simulink model "FOCsimulation"  (R2023b)
settings: Solver=VariableStepAuto  StartTime=0.0  StopTime=12  RelTol=1e-3
values from neighbouring files (symbols this model uses):
  acceleration = 20000/PU_System.N_base    [FOC_Script.m]    (also in Motor_script.m)
  PI_params = mcb.internal.SetControllerParameters(pmsm,inverter,PU_System,T_pwm,2*Ts,Ts_speed)    [FOC_Script.m]    (also in Motor_script.m)
  Speed_openLoop_PU = 0.1    [FOC_Script.m]    (also in Motor_script.m)
  T_Ref_openLoop = 1    [FOC_Script.m]    (also in Motor_script.m)
  Ts = T_pwm    (= 0.0001)    [FOC_Script.m]    (also in Motor_script.m = 3.33333333333e-05)
  Ts_motor = T_pwm/2    (= 5e-05)    [FOC_Script.m]    (also in Motor_script.m = 1.66666666667e-05)
  Ts_speed = 30*Ts    (= 0.003)    [FOC_Script.m]    (also in Motor_script.m = 0.001)
undefined symbols (not defined in the file or in its folder): inverter, pmsm, PU_System, sigbuilder_block, target
libraries: mcbcontrolslib x11, slpidlib x3, mcbpositiondecoderlib x2, simulink x1, dspsrcs4 x1, mcbplantlib x1, autolibpmsmexterior x1
(part 2 of 2)

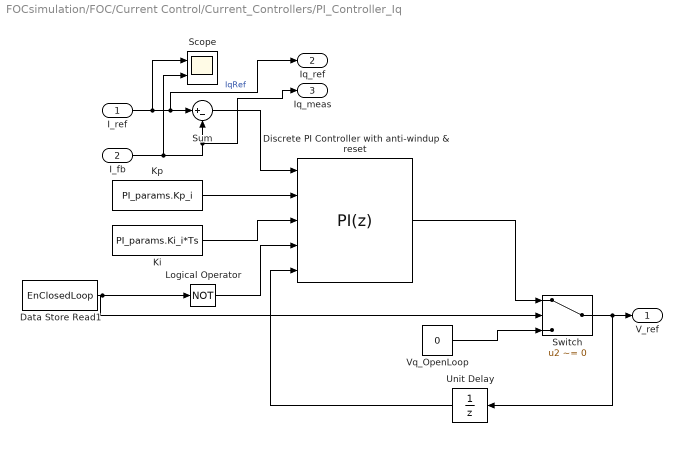
== system FOCsimulation/FOC/Current Control/Current_Controllers/PI_Controller_Iq ==
  I_ref : Inport
  I_fb : Inport  Port=2
  Data Store Read1 : DataStoreRead  DataStoreName=EnClosedLoop  IndexOptions=Index vector (dialog)  Indices=1  OutputSizes=1
  Discrete PI Controller with anti-windup & reset : slpidlib/PID Controller  Controller=PI  Form=Parallel  TimeDomain=Discrete-time  UseExternalTs=off  SampleTime=-1  IntegratorMethod=Forward Euler  FilterMethod=Forward Euler  ControllerParametersSource=external  P=1  I=1  UseKiTs=on  D=0  N=100  UseFilter=on  TunerSelectOption=Transfer Function Based (PID Tuner App)  InitialConditionSource=external  InitialConditionForIntegrator=0  InitialConditionForFilter=0  DifferentiatorICPrevScaledInput=0  ExternalReset=level  TrackingMode=off  Kt=1  LimitOutput=on  SatLimitsSource=internal  UpperSaturationLimit=1  LowerSaturationLimit=-1  LinearizeAsGain=on  AntiWindupMode=clamping  Kb=1  LimitIntegrator=off  UpperIntegratorSaturationLimit=inf  LowerIntegratorSaturationLimit=-inf  RndMeth=Simplest  POutMin=[]  POutMax=[]  IOutMin=[]  IOutMax=[]  DOutMin=[]  DOutMax=[]  NOutMin=[]  NOutMax=[]  SumOutMin=[]  SumOutMax=[]  SaturationOutDataTypeStr=Inherit: Inherit via back propagation  SaturationOutMin=[]  SaturationOutMax=[]  PParamMin=[]  PParamMax=[]  IParamMin=[]  IParamMax=[]  DParamMin=[]  DParamMax=[]  NParamMin=[]  NParamMax=[]  KbParamMin=[]  KbParamMax=[]  KtParamMin=[]  KtParamMax=[]  KbOutMin=[]  KbOutMax=[]  KtOutMin=[]  KtOutMax=[]  IntegratorOutMin=[]  IntegratorOutMax=[]  FilterOutMin=[]  FilterOutMax=[]  SumI1OutMin=[]  SumI1OutMax=[]  SumI2OutMin=[]  SumI2OutMax=[]  SumI3OutMin=[]  SumI3OutMax=[]  SumI4OutMin=[]  SumI4OutMax=[]  SumDOutMin=[]  SumDOutMax=[]  DifferentiatorOutMin=[]  DifferentiatorOutMax=[]  FilterDiffOutCoefMin=[]  FilterDiffOutCoefMax=[]  ReciprocalOutMin=[]  ReciprocalOutMax=[]  SumDenOutMin=[]  SumDenOutMax=[]  SumNumOutMin=[]  SumNumOutMax=[]  DivideOutMin=[]  DivideOutMax=[]  UdiffTsProdOutMin=[]  UdiffTsProdOutMax=[]  NTsProdOutMin=[]  NTsProdOutMax=[]  UintegralTsProdOutMin=[]  UintegralTsProdOutMax=[]  UngainTsProdOutMin=[]  UngainTsProdOutMax=[]  ClampingZeroOutDataTypeStr=Inherit: Inherit via back propagation  ClampingZeroOutMin=[]  ClampingZeroOutMax=[]  FilterDenConstantOutDataTypeStr=Inherit: Inherit via back propagation  FilterDenConstantOutMin=[]  FilterDenConstantOutMax=[]  PCopyOutDataTypeStr=Inherit: Inherit via back propagation  PCopyOutMin=[]  PCopyOutMax=[]  NCopyOutDataTypeStr=Inherit: Inherit via back propagation  NCopyOutMin=[]  NCopyOutMax=[]  IntegratorContinuousStateAttributes=''  IntegratorStateMustResolveToSignalObject=off  IntegratorRTWStateStorageClass=Auto  FilterContinuousStateAttributes=''  FilterStateMustResolveToSignalObject=off  FilterRTWStateStorageClass=Auto  ParallelPVariant=ExternalParameters  IdealPVariant=Disabled  IVariant=ExternalParameters  DVariant=Disabled  IntegratorVariant=Discrete  SatVariant=Enabled  AWVariant=DiscClampingParallel  PCopyVariant=Disabled  TRVariant=Disabled  FdbkBlocksVariant=Forward  IdealPFdbkVariant=Disabled  SatFdbkVariant=Disabled  DerivativeFilterVariant=Disabled  NVariant=Disabled  NCopyVariant=Disabled_SignalSpec  FilterICVariant=Disabled  IntegratorICVariant=ExternalICs  ExternalResetVariant=ExternalReset  TRSumVariant=Passthrough  SumFdbkVariant=Disabled  SumVariant=Sum_PI  TsampFilterVariant=InternalTs  TsampNgainVariant=Passthrough  TsampIntegralVariant=Disabled_SignalSpec  ExternalSaturationOutDataTypeStr=Inherit: Same as second input
      settings: LibrarySourceBlock=mcbcontrolslib/PI Controller
  Ki : Constant  Value=PI_params.Ki_i*Ts  OutDataTypeStr=dataType  SampleTime=-1
  Kp : Constant  Value=PI_params.Kp_i  OutDataTypeStr=dataType  SampleTime=-1
  Logical Operator : Logic  Operator=NOT  IconShape=distinctive  AllPortsSameDT=off  OutDataTypeStr=boolean
  Scope : Scope  NumInputPorts=2
  Sum : Sum  Inputs=|+-  OutDataTypeStr=Inherit: Same as first input
  Switch : Switch  Criteria=u2 ~= 0  RndMeth=Simplest  SaturateOnIntegerOverflow=off  InputSameDT=off
  Unit Delay : UnitDelay  SampleTime=-1  HasFrameUpgradeWarning=on
  Vq_OpenLoop : Constant  Value=0  OutDataTypeStr=dataType  SampleTime=-1
  V_ref : Outport  VectorParamsAs1DForOutWhenUnconnected=off
  Iq_ref : Outport  Port=2  VectorParamsAs1DForOutWhenUnconnected=off
  Iq_meas : Outport  Port=3  VectorParamsAs1DForOutWhenUnconnected=off
  wires:
  Switch/1 -> V_ref/1, Unit Delay/1
  I_fb/1 -> Scope/2, Iq_meas/1, Sum/2
  Sum/1 -> Discrete PI Controller with anti-windup & reset/1
  Kp/1 -> Discrete PI Controller with anti-windup & reset/2
  I_ref/1 -> Scope/1, Iq_ref/1, Sum/1  "IqRef"
  Ki/1 -> Discrete PI Controller with anti-windup & reset/3
  Logical Operator/1 -> Discrete PI Controller with anti-windup & reset/4
  Unit Delay/1 -> Discrete PI Controller with anti-windup & reset/5
  Discrete PI Controller with anti-windup & reset/1 -> Switch/1
  Vq_OpenLoop/1 -> Switch/3
  Data Store Read1/1 -> Switch/2, Logical Operator/1

== system FOCsimulation/FOC/Speed Control/Speed_Ref_Selector/Absolute value ==
  Speed_Ref : Inport
  Rate Limiter : RateLimiter  RisingSlewLimit=acceleration  FallingSlewLimit=-acceleration  SampleTimeMode=inherited  InitialCondition=Speed_openLoop_PU
  Rate Limiter1 : RateLimiter  RisingSlewLimit=acceleration  FallingSlewLimit=-acceleration  SampleTimeMode=inherited  InitialCondition=-Speed_openLoop_PU
  Switch : Switch  SaturateOnIntegerOverflow=off  InputSameDT=off
  Out1 : Outport
  wires:
  Switch/1 -> Out1/1
  Rate Limiter/1 -> Switch/1
  Rate Limiter1/1 -> Switch/3
  Speed_Ref/1 -> Rate Limiter/1, Rate Limiter1/1, Switch/2

== system FOCsimulation/FOC/Current Control/Calculate position and speed/Flux Observer/DC component removal ==
  SigIN : Inport
  IIR Filter : mcbcontrolslib/IIR Filter  VariantControl=Low Pass Filter  VariantSelect=Low-pass  Filter_constant=0.005*(Ts/50e-6)  advancedSettings=off  Ts=50e-6  cutOff_freq=32.1525
  Sum6 : Sum  Inputs=|+-  RndMeth=Simplest  OutDataTypeStr=Inherit: Same as first input
  SigOUT : Outport
  wires:
  IIR Filter/1 -> Sum6/2
  SigIN/1 -> IIR Filter/1, Sum6/1
  Sum6/1 -> SigOUT/1
